simulink model "FMS"  (R2018b)
settings: configuration reference "fms_config" (kept outside this file)
values from neighbouring files (symbols this model uses):
  FMS_EXPORT = Simulink.Parameter(FMS_EXPORT_VALUE)    [fms_model_init.m]
  FMS_PARAM = Simulink.Parameter(FMS_PARAM_VALUE)    [fms_model_init.m]
undefined symbols (not defined in the file or in its folder): actuator_cmd, ax_cmd, ay_cmd, az_cmd, cmd_mask, ControlMode, ctrl_mode, DiscIntNeverNeededParam, ext_state, FMS_Cmd, FMS_CONST, home, mode, p_cmd, phi_cmd, PilotMode, psi_rate_cmd, q_cmd, r_cmd, reset, state, status, theta_cmd, throttle_cmd, timestamp, u_cmd, v_cmd, VehicleState, VehicleStatus, VTOLState, w_cmd, wp_consume, wp_current
libraries: simulink x141, FMT_Model_Lib x120, hdlsllib x13
(part 8 of 12)

== system FMS/FMS Commander/Commander/Arm/MC_Mode/SubMode/Takeoff/Climb Speed/TD/fhan  ==
  v1 : Inport
  v2 : Inport  Port=2
  Abs : Abs
  Add{,1..3,5..6} (6 alike) : Sum  OutDataTypeStr=Inherit: Same as first input
  Add4 : Sum  Inputs=-++
  Divide : Product  Inputs=*/
  Gain : Gain  Gain=8
  Gain1 : Gain  Gain=0.5  OutDataTypeStr=Inherit: Same as input
  Gain2 : Gain  Gain=0.5  OutDataTypeStr=Inherit: Same as input
  Gain3 : Gain  Gain=0.5  OutDataTypeStr=Inherit: Same as input
  Gain4 : Gain  Gain=-1  OutDataTypeStr=Inherit: Same as input
  Multiply{,1..3} (4 alike) : Product  OutDataTypeStr=Inherit: Same as first input
  Multiply4 : Product  OutDataTypeStr=single
  Multiply5 : Product  Inputs=3
  Multiply6 : Product  OutDataTypeStr=single
  Sign{,1..6} (7 alike) : Signum
  Sqrt : Sqrt  SaturateOnIntegerOverflow=on
  Square : Math  Operator=square  SaturateOnIntegerOverflow=on
  Subtract{,1..5} (6 alike) : Sum  Inputs=+-  OutDataTypeStr=Inherit: Same as first input
  Subtract6 : Sum  Inputs=-+  OutDataTypeStr=Inherit: Same as first input
  const : Constant  Value=r0  OutDataTypeStr=single
  const1 : Constant  Value=h0  OutDataTypeStr=single
  fhan : Outport
  wires:
  v1/1 -> Add/1
  Sign/1 -> Multiply3/1
  Gain2/1 -> Multiply4/2  "sy"
  v2/1 -> Multiply1/1
  Gain3/1 -> Multiply5/3  "sa"
  Subtract/1 -> Gain1/1
  Subtract6/1 -> fhan/1
  Sign2/1 -> Subtract2/2
  Sign4/1 -> Subtract4/2
  Abs/1 -> Gain/1
  Add4/1 -> Multiply4/1
  Sign5/1 -> Subtract5/2
  Sqrt/1 -> Subtract/1  "a1"
  Subtract3/1 -> Sign4/1
  Add1/1 -> Multiply2/1
  Subtract1/1 -> Sign2/1
  Divide/1 -> Subtract5/1
  Multiply3/1 -> Add2/1
  Gain/1 -> Add1/2
  const/1 -> Multiply6/2, Gain4/1, Multiply/1
  Add3/1 -> Sign1/1
  Subtract5/1 -> Multiply5/2
  Multiply4/1 -> Add5/2
  const1/1 -> Multiply1/2, Square/1
  Add5/1 -> Sign6/1, Sign5/1, Divide/1, Subtract3/1, Add6/1  "a"
  Multiply1/1 -> Add4/3, Add2/2, Add/2  "a0"
  Add/1 -> Subtract1/1, Add3/1, Add4/2, Sign/1, Abs/1  "y"
  Subtract2/1 -> Gain2/1
  Add2/1 -> Add4/1, Add5/1  "a2"
  Subtract4/1 -> Gain3/1
  Gain4/1 -> Multiply5/1
  Multiply5/1 -> Subtract6/2
  Sign6/1 -> Multiply6/1
  Sign3/1 -> Subtract4/1
  Add6/1 -> Sign3/1
  Multiply/1 -> Subtract/2, Divide/2, Subtract3/2, Add6/2, Subtract1/2, Add3/2, Add1/1, Multiply2/2  "d"
  Multiply6/1 -> Subtract6/1
  Gain1/1 -> Multiply3/2
  Square/1 -> Multiply/2
  Multiply2/1 -> Sqrt/1
  Sign1/1 -> Subtract2/1

== system FMS/FMS Commander/Commander/Arm/BackwardTrans_Mode/Position Command/Controller/Hold Control/Lateral_Acceleration/L1_Lateral_Acceleration/Included Angle ==
  vec1 : Inport
  vec2 : Inport  Port=2
  2D Cross Product : FMT_Model_Lib/Math/2D Cross Product
      settings: SourceProductName=FMT Toolbox
  Acos : Trigonometry  Operator=acos
  Constant4 : Constant  OutDataTypeStr=single
  Demux : Demux  Outputs=2
  Demux1 : Demux  Outputs=2
  Dot Product : DotProduct  InputSameDT=on  OutDataTypeStr=Inherit: Inherit via internal rule
  Multiply : Product
  Mux : Mux  Inputs=2
  Mux1 : Mux  Inputs=2
  Sign1 : Signum
  Switch2 : Switch  Criteria=u2 ~= 0
  Vector Normalize : FMT_Model_Lib/Math/Vector Normalize
      settings: SourceProductName=FMT Toolbox
  Vector Normalize1 : FMT_Model_Lib/Math/Vector Normalize
      settings: SourceProductName=FMT Toolbox
  angle_rad : Outport
  wires:
  Switch2/1 -> Multiply/2
  Acos/1 -> Multiply/1
  Mux/1 -> Vector Normalize1/1
  vec2/1 -> Demux/1
  Constant4/1 -> Switch2/3
  Demux/1 -> Mux/2
  vec1/1 -> Demux1/1
  Multiply/1 -> angle_rad/1
  2D Cross Product/1 -> Sign1/1
  Vector Normalize/1 -> 2D Cross Product/2, Dot Product/1
  Demux/2 -> Mux/1
  Vector Normalize1/1 -> 2D Cross Product/1, Dot Product/2
  Sign1/1 -> Switch2/2, Switch2/1
  Demux1/2 -> Mux1/1
  Mux1/1 -> Vector Normalize/1
  Demux1/1 -> Mux1/2
  Dot Product/1 -> Acos/1

== system FMS/FMS Commander/Commander/Arm/BackwardTrans_Mode/Position Command/Controller/Hold Control/Velocity_Controller/Error/Bus_Select ==
  INS_Out : Inport
  Bus Selector1 : BusSelector  OutputSignals=vn,ve
  Bus Selector2 : BusSelector  OutputSignals=psi
  Constant : Constant  Value=0  OutDataTypeStr=single
  Multiply : Product  Multiplication=Matrix(*)
  Mux2 : Mux  Inputs=3
  Psi To DCM : FMT_Model_Lib/Transformation/Psi To DCM
      settings: SourceProductName=FMT Toolbox
  Selector : Selector  InputPortWidth=3  IndexOptions=Index vector (dialog)  Indices=2  OutputSizes=1
  v_est_C_mPs : Outport
  wires:
  Psi To DCM/1 -> Multiply/1
  Bus Selector2/1 -> Psi To DCM/1  "<psi>"
  Constant/1 -> Mux2/3  "<velD>"
  Mux2/1 -> Multiply/2
  Bus Selector1/2 -> Mux2/2  "<ve>"
  Bus Selector1/1 -> Mux2/1  "<vn>"
  INS_Out/1 -> Bus Selector2/1, Bus Selector1/1
  Multiply/1 -> Selector/1
  Selector/1 -> v_est_C_mPs/1

== system FMS/FMS Commander/Commander/Arm/BackwardTrans_Mode/Position Command/Controller/Hold Control/Velocity_Controller/PID_Controller/D_Control ==
  err : Inport
  reset : Inport  Port=2
  DT Filter : FMT_Model_Lib/Filter/DT Filter  fc=10
      settings: SourceProductName=FMT Toolbox
  Multiply : Product  OutDataTypeStr=Inherit: Same as first input
  Saturation : Saturate  UpperLimit=max_d  LowerLimit=min_d
  kd : Constant  Value=kd  OutDataTypeStr=single
  d_out : Outport
  wires:
  err/1 -> DT Filter/1
  kd/1 -> Multiply/1
  Multiply/1 -> Saturation/1
  Saturation/1 -> d_out/1
  reset/1 -> DT Filter/2
  DT Filter/1 -> Multiply/2

== system FMS/FMS Commander/Commander/Arm/BackwardTrans_Mode/Position Command/Controller/Hold Control/Velocity_Controller/PID_Controller/I_Control ==
  err : Inport
  reset : Inport  Port=2
  Constant : Constant  Value=0  OutDataTypeStr=single
  Discrete-Time Integrator : DiscreteIntegrator  ExternalReset=level  InitialConditionSource=external  SampleTime=-1  LimitOutput=on  UpperSaturationLimit=max_i  LowerSaturationLimit=min_i  ICPrevOutput=DiscIntNeverNeededParam  ICPrevScaledInput=DiscIntNeverNeededParam
  Multiply : Product  OutDataTypeStr=Inherit: Same as first input
  ki : Constant  Value=ki  OutDataTypeStr=single
  i_out : Outport
  wires:
  err/1 -> Multiply/2
  Multiply/1 -> Discrete-Time Integrator/1
  reset/1 -> Discrete-Time Integrator/2
  Constant/1 -> Discrete-Time Integrator/3
  Discrete-Time Integrator/1 -> i_out/1
  ki/1 -> Multiply/1

== system FMS/FMS Commander/Commander/Arm/BackwardTrans_Mode/Position Command/Controller/Hold Control/Velocity_Controller/PID_Controller/P_Control ==
  err : Inport
  Multiply : Product  OutDataTypeStr=Inherit: Same as first input
  kp : Constant  Value=kp  OutDataTypeStr=single
  p_out : Outport
  wires:
  err/1 -> Multiply/2
  kp/1 -> Multiply/1
  Multiply/1 -> p_out/1

== system FMS/FMS Commander/Commander/Arm/FW_Mode/Assist/Altitude/Altitude Command/Controller/Hold Control/Bus_Selection ==
  FMS_In : Inport
  Bus Selector2 : BusSelector  OutputSignals=INS_Out.h_R
  Gain : Gain  Gain=-1
  z_R_m : Outport
  wires:
  Gain/1 -> z_R_m/1
  Bus Selector2/1 -> Gain/1  "<h_R>"
  FMS_In/1 -> Bus Selector2/1

== system FMS/FMS Commander/Commander/Arm/FW_Mode/Assist/Altitude/Altitude Command/Controller/Move Control/DeadZone ==
  u : Inport
  Dead Zone : DeadZone  LowerValue=-th  UpperValue=th  SaturateOnIntegerOverflow=on
  Gain : Gain  Gain=1/(1-th)
  y : Outport
  wires:
  Gain/1 -> y/1
  Dead Zone/1 -> Gain/1
  u/1 -> Dead Zone/1

== system FMS/FMS Commander/Commander/Arm/FW_Mode/Assist/Altitude/Altitude Command/Controller/Move Control/TD1 ==
  v : Inport
  Integrator : DiscreteIntegrator  SampleTime=-1  ICPrevOutput=DiscIntNeverNeededParam  ICPrevScaledInput=DiscIntNeverNeededParam
  Integrator1 : DiscreteIntegrator  SampleTime=-1  ICPrevOutput=DiscIntNeverNeededParam  ICPrevScaledInput=DiscIntNeverNeededParam
  Subtract : Sum  Inputs=+-
  "fhan " : Subsystem  mask{r0=8*9.806, h0=0.05}
      mask DialogControl ParameterGroupVar Prompt: fhan(v1,v2,r0,h0)
  v1 : Outport
  wires:
  Integrator1/1 -> v1/1, Subtract/1
  v/1 -> Subtract/2
  Integrator/1 -> "fhan "/2(v2), Integrator1/1  "v2"
  Subtract/1 -> "fhan "/1(v1)
  "fhan "/1(fhan) -> Integrator/1

== system FMS/FMS Commander/Commander/Arm/FW_Mode/Assist/Altitude/Altitude Command/Controller/TD/fhan  ==
  v1 : Inport
  v2 : Inport  Port=2
  Abs : Abs
  Add{,1..3,5..6} (6 alike) : Sum  OutDataTypeStr=Inherit: Same as first input
  Add4 : Sum  Inputs=-++
  Divide : Product  Inputs=*/
  Gain : Gain  Gain=8
  Gain1 : Gain  Gain=0.5  OutDataTypeStr=Inherit: Same as input
  Gain2 : Gain  Gain=0.5  OutDataTypeStr=Inherit: Same as input
  Gain3 : Gain  Gain=0.5  OutDataTypeStr=Inherit: Same as input
  Gain4 : Gain  Gain=-1  OutDataTypeStr=Inherit: Same as input
  Multiply{,1..3} (4 alike) : Product  OutDataTypeStr=Inherit: Same as first input
  Multiply4 : Product  OutDataTypeStr=single
  Multiply5 : Product  Inputs=3
  Multiply6 : Product  OutDataTypeStr=single
  Sign{,1..6} (7 alike) : Signum
  Sqrt : Sqrt  SaturateOnIntegerOverflow=on
  Square : Math  Operator=square  SaturateOnIntegerOverflow=on
  Subtract{,1..5} (6 alike) : Sum  Inputs=+-  OutDataTypeStr=Inherit: Same as first input
  Subtract6 : Sum  Inputs=-+  OutDataTypeStr=Inherit: Same as first input
  const : Constant  Value=r0  OutDataTypeStr=single
  const1 : Constant  Value=h0  OutDataTypeStr=single
  fhan : Outport
  wires:
  Sign1/1 -> Subtract2/1
  Multiply2/1 -> Sqrt/1
  Square/1 -> Multiply/2
  Gain1/1 -> Multiply3/2
  Multiply6/1 -> Subtract6/1
  Multiply/1 -> Multiply2/2, Add1/1, Add3/2, Subtract1/2, Add6/2, Subtract3/2, Divide/2, Subtract/2  "d"
  Add6/1 -> Sign3/1
  Sign3/1 -> Subtract4/1
  Sign6/1 -> Multiply6/1
  Multiply5/1 -> Subtract6/2
  Gain4/1 -> Multiply5/1
  Subtract4/1 -> Gain3/1
  Add2/1 -> Add5/1, Add4/1  "a2"
  Subtract2/1 -> Gain2/1
  Add/1 -> Abs/1, Sign/1, Add4/2, Add3/1, Subtract1/1  "y"
  Multiply1/1 -> Add/2, Add2/2, Add4/3  "a0"
  Add5/1 -> Add6/1, Subtract3/1, Divide/1, Sign5/1, Sign6/1  "a"
  const1/1 -> Square/1, Multiply1/2
  Multiply4/1 -> Add5/2
  Subtract5/1 -> Multiply5/2
  Add3/1 -> Sign1/1
  const/1 -> Multiply/1, Gain4/1, Multiply6/2
  Gain/1 -> Add1/2
  Multiply3/1 -> Add2/1
  Divide/1 -> Subtract5/1
  Subtract1/1 -> Sign2/1
  Add1/1 -> Multiply2/1
  Subtract3/1 -> Sign4/1
  Sqrt/1 -> Subtract/1  "a1"
  Sign5/1 -> Subtract5/2
  Add4/1 -> Multiply4/1
  Abs/1 -> Gain/1
  Sign4/1 -> Subtract4/2
  Sign2/1 -> Subtract2/2
  Subtract6/1 -> fhan/1
  Subtract/1 -> Gain1/1
  Gain3/1 -> Multiply5/3  "sa"
  v2/1 -> Multiply1/1
  Gain2/1 -> Multiply4/2  "sy"
  Sign/1 -> Multiply3/1
  v1/1 -> Add/1

== system FMS/FMS Commander/Commander/Arm/FW_Mode/Assist/Position/Altitude Command/Controller/Hold Control/Bus_Selection ==
  FMS_In : Inport
  Bus Selector2 : BusSelector  OutputSignals=INS_Out.h_R
  Gain : Gain  Gain=-1
  z_R_m : Outport
  wires:
  Gain/1 -> z_R_m/1
  Bus Selector2/1 -> Gain/1  "<h_R>"
  FMS_In/1 -> Bus Selector2/1

== system FMS/FMS Commander/Commander/Arm/FW_Mode/Assist/Position/Altitude Command/Controller/Move Control/DeadZone ==
  u : Inport
  Dead Zone : DeadZone  LowerValue=-th  UpperValue=th  SaturateOnIntegerOverflow=on
  Gain : Gain  Gain=1/(1-th)
  y : Outport
  wires:
  Gain/1 -> y/1
  Dead Zone/1 -> Gain/1
  u/1 -> Dead Zone/1

== system FMS/FMS Commander/Commander/Arm/FW_Mode/Assist/Position/Altitude Command/Controller/Move Control/TD1 ==
  v : Inport
  Integrator : DiscreteIntegrator  SampleTime=-1  ICPrevOutput=DiscIntNeverNeededParam  ICPrevScaledInput=DiscIntNeverNeededParam
  Integrator1 : DiscreteIntegrator  SampleTime=-1  ICPrevOutput=DiscIntNeverNeededParam  ICPrevScaledInput=DiscIntNeverNeededParam
  Subtract : Sum  Inputs=+-
  "fhan " : Subsystem  mask{r0=8*9.806, h0=0.05}
      mask DialogControl ParameterGroupVar Prompt: fhan(v1,v2,r0,h0)
  v1 : Outport
  wires:
  Integrator1/1 -> v1/1, Subtract/1
  v/1 -> Subtract/2
  Integrator/1 -> "fhan "/2(v2), Integrator1/1  "v2"
  Subtract/1 -> "fhan "/1(v1)
  "fhan "/1(fhan) -> Integrator/1

== system FMS/FMS Commander/Commander/Arm/FW_Mode/Assist/Position/Altitude Command/Controller/TD/fhan  ==
  v1 : Inport
  v2 : Inport  Port=2
  Abs : Abs
  Add{,1..3,5..6} (6 alike) : Sum  OutDataTypeStr=Inherit: Same as first input
  Add4 : Sum  Inputs=-++
  Divide : Product  Inputs=*/
  Gain : Gain  Gain=8
  Gain1 : Gain  Gain=0.5  OutDataTypeStr=Inherit: Same as input
  Gain2 : Gain  Gain=0.5  OutDataTypeStr=Inherit: Same as input
  Gain3 : Gain  Gain=0.5  OutDataTypeStr=Inherit: Same as input
  Gain4 : Gain  Gain=-1  OutDataTypeStr=Inherit: Same as input
  Multiply{,1..3} (4 alike) : Product  OutDataTypeStr=Inherit: Same as first input
  Multiply4 : Product  OutDataTypeStr=single
  Multiply5 : Product  Inputs=3
  Multiply6 : Product  OutDataTypeStr=single
  Sign{,1..6} (7 alike) : Signum
  Sqrt : Sqrt  SaturateOnIntegerOverflow=on
  Square : Math  Operator=square  SaturateOnIntegerOverflow=on
  Subtract{,1..5} (6 alike) : Sum  Inputs=+-  OutDataTypeStr=Inherit: Same as first input
  Subtract6 : Sum  Inputs=-+  OutDataTypeStr=Inherit: Same as first input
  const : Constant  Value=r0  OutDataTypeStr=single
  const1 : Constant  Value=h0  OutDataTypeStr=single
  fhan : Outport
  wires:
  Sign1/1 -> Subtract2/1
  Multiply2/1 -> Sqrt/1
  Square/1 -> Multiply/2
  Gain1/1 -> Multiply3/2
  Multiply6/1 -> Subtract6/1
  Multiply/1 -> Multiply2/2, Add1/1, Add3/2, Subtract1/2, Add6/2, Subtract3/2, Divide/2, Subtract/2  "d"
  Add6/1 -> Sign3/1
  Sign3/1 -> Subtract4/1
  Sign6/1 -> Multiply6/1
  Multiply5/1 -> Subtract6/2
  Gain4/1 -> Multiply5/1
  Subtract4/1 -> Gain3/1
  Add2/1 -> Add5/1, Add4/1  "a2"
  Subtract2/1 -> Gain2/1
  Add/1 -> Abs/1, Sign/1, Add4/2, Add3/1, Subtract1/1  "y"
  Multiply1/1 -> Add/2, Add2/2, Add4/3  "a0"
  Add5/1 -> Add6/1, Subtract3/1, Divide/1, Sign5/1, Sign6/1  "a"
  const1/1 -> Square/1, Multiply1/2
  Multiply4/1 -> Add5/2
  Subtract5/1 -> Multiply5/2
  Add3/1 -> Sign1/1
  const/1 -> Multiply/1, Gain4/1, Multiply6/2
  Gain/1 -> Add1/2
  Multiply3/1 -> Add2/1
  Divide/1 -> Subtract5/1
  Subtract1/1 -> Sign2/1
  Add1/1 -> Multiply2/1
  Subtract3/1 -> Sign4/1
  Sqrt/1 -> Subtract/1  "a1"
  Sign5/1 -> Subtract5/2
  Add4/1 -> Multiply4/1
  Abs/1 -> Gain/1
  Sign4/1 -> Subtract4/2
  Sign2/1 -> Subtract2/2
  Subtract6/1 -> fhan/1
  Subtract/1 -> Gain1/1
  Gain3/1 -> Multiply5/3  "sa"
  v2/1 -> Multiply1/1
  Gain2/1 -> Multiply4/2  "sy"
  Sign/1 -> Multiply3/1
  v1/1 -> Add/1

== system FMS/FMS Commander/Commander/Arm/FW_Mode/Assist/Position/Position Command/Controller/Hold Control/Fly_Direction ==
  FMS_In : Inport
  Bus Selector2 : BusSelector  OutputSignals=INS_Out.vn,INS_Out.ve,INS_Out.vd
  Bus Selector3 : BusSelector  OutputSignals=INS_Out.quat
  Multiply : Product  Multiplication=Matrix(*)
  Mux : Mux  Inputs=3
  Quaternion To DCM : FMT_Model_Lib/Quaternion/Quaternion To DCM
      settings: SourceProductName=FMT Toolbox
  Selector : Selector  InputPortWidth=3  IndexOptions=Index vector (dialog)  Indices=1  OutputSizes=1
  Sign : Signum
  sign : Outport
  wires:
  Bus Selector3/1 -> Quaternion To DCM/1  "<quat>"
  Multiply/1 -> Selector/1
  Bus Selector2/3 -> Mux/3  "<vd>"
  FMS_In/1 -> Bus Selector3/1, Bus Selector2/1
  Sign/1 -> sign/1
  Mux/1 -> Multiply/2
  Quaternion To DCM/1 -> Multiply/1
  Bus Selector2/2 -> Mux/2  "<ve>"
  Bus Selector2/1 -> Mux/1  "<vn>"
  Selector/1 -> Sign/1  "Vu"

== system FMS/FMS Commander/Commander/Arm/FW_Mode/Assist/Position/Position Command/Controller/Hold Control/L1_Reference_WP ==
  c : Inport
  p_0 : Inport  Port=2
  n : Inport  Port=3
  L1 : Inport  Port=4
  Compare To Zero : simulink/Logic and Bit Operations/Compare To Zero  relop=>  OutDataTypeStr=boolean
  OutRegionRefWP : MATLAB Function  TreatAsAtomicUnit=on
  SearchL1RefWP : MATLAB Function  TreatAsAtomicUnit=on
  Switch : Switch  Criteria=u2 > Threshold
  L1_WP : Outport
  wires:
  c/1 -> OutRegionRefWP/1(c), SearchL1RefWP/1(c)
  p_0/1 -> OutRegionRefWP/2(p0), SearchL1RefWP/2(p0)
  n/1 -> OutRegionRefWP/3(n), SearchL1RefWP/3(n)
  L1/1 -> SearchL1RefWP/4(L1)
  SearchL1RefWP/1(P) -> Switch/1
  SearchL1RefWP/2(t) -> Compare To Zero/1
  Compare To Zero/1 -> Switch/2
  OutRegionRefWP/1(P) -> Switch/3
  Switch/1 -> L1_WP/1

== system FMS/FMS Commander/Commander/Arm/FW_Mode/Assist/Position/Position Command/Controller/Hold Control/Lateral_Acceleration ==
  p_vehicle : Inport
  L1_WP : Inport  Port=2
  L1 : Inport  Port=3
  Vg : Inport  Port=4
  L1_Lateral_Acceleration : Subsystem
  Subtract : Sum  Inputs=+-
  ay_cmd_mPs2 : Outport
  wires:
  L1_WP/1 -> Subtract/1
  p_vehicle/1 -> Subtract/2
  L1/1 -> L1_Lateral_Acceleration/1(L1)
  Vg/1 -> L1_Lateral_Acceleration/2(Vg)
  Subtract/1 -> L1_Lateral_Acceleration/3(l1_path)
  L1_Lateral_Acceleration/1(l1_a_cmd) -> ay_cmd_mPs2/1

== system FMS/FMS Commander/Commander/Arm/FW_Mode/Assist/Position/Position Command/Controller/Hold Control/Path_Ray ==
  note: p(t) = p0 + t*n
  FMS_In : Inport
  Bus Selector1 : BusSelector  OutputSignals=INS_Out.x_R,INS_Out.y_R
  Bus Selector2 : BusSelector  OutputSignals=INS_Out.vn,INS_Out.ve
  Bus Selector3 : BusSelector  Commented=on  OutputSignals=INS_Out.psi
  Constant : Constant  Commented=on  Value=[1;0;0]  VectorParams1D=off  OutDataTypeStr=single
  Multiply : Product  Commented=on  Multiplication=Matrix(*)
  Mux : Mux  Inputs=2
  Mux1 : Mux  Inputs=2
  Psi To DCM : FMT_Model_Lib/Transformation/Psi To DCM  Commented=on
      settings: SourceProductName=FMT Toolbox
  Selector : Selector  Commented=on  InputPortWidth=3  IndexOptions=Index vector (dialog)  Indices=[1 2]  OutputSizes=1
  Terminator : Terminator  Commented=on
  Transpose : Math  Commented=on  Operator=transpose  SaturateOnIntegerOverflow=on
  Vector Normalize : FMT_Model_Lib/Math/Vector Normalize
      settings: SourceProductName=FMT Toolbox
  start_vel : Delay  DelayLength=1  InitialConditionSource=Input port
      settings: InputPortMap=u0,p4
  start_wp : Delay  DelayLength=1  InitialConditionSource=Input port
      settings: InputPortMap=u0,p4
  p_vehicle : Outport
  p_0 : Outport  Port=2
  n : Outport  Port=3
  wires:
  Bus Selector2/2 -> Mux1/2  "<ve>"
  Bus Selector1/2 -> Mux/2  "<y_R>"
  Mux/1 -> p_vehicle/1, start_wp/2
  start_wp/1 -> p_0/1, start_wp/1
  Bus Selector1/1 -> Mux/1  "<x_R>"
  start_vel/1 -> Vector Normalize/1, start_vel/1
  Bus Selector2/1 -> Mux1/1  "<vn>"
  Vector Normalize/1 -> n/1
  FMS_In/1 -> Bus Selector3/1, Bus Selector2/1, Bus Selector1/1
  Mux1/1 -> start_vel/2
  Bus Selector3/1 -> Psi To DCM/1  "<psi>"
  Psi To DCM/1 -> Transpose/1
  Transpose/1 -> Multiply/1
  Constant/1 -> Multiply/2
  Multiply/1 -> Selector/1
  Selector/1 -> Terminator/1

== system FMS/FMS Commander/Commander/Arm/FW_Mode/Assist/Position/Position Command/Controller/Hold Control/Velocity_Controller ==
  FMS_In : Inport
  Bus Selector : BusSelector  OutputSignals=INS_Out
  Constant : Constant  Value=0  OutDataTypeStr=Inherit: Inherit via back propagation
  Error : Subsystem
  PID_Controller : Subsystem
  ay_cmd_B_rad : Outport
  wires:
  FMS_In/1 -> Bus Selector/1
  Error/1(v_err_C_mPs) -> PID_Controller/1(uv_err_C_mPs)
  PID_Controller/1(accel_cmd_C) -> ay_cmd_B_rad/1
  Bus Selector/1 -> Error/1(INS_Out)  "<INS_Out>"
  Constant/1 -> PID_Controller/2(reset)

== system FMS/FMS Commander/Commander/Arm/FW_Mode/Assist/Position/Position Command/Controller/Move Control/DeadZone1 ==
  u : Inport
  Dead Zone : DeadZone  LowerValue=-th  UpperValue=th  SaturateOnIntegerOverflow=on
  Gain : Gain  Gain=1/(1-th)
  y : Outport
  wires:
  u/1 -> Dead Zone/1
  Dead Zone/1 -> Gain/1
  Gain/1 -> y/1

== system FMS/FMS Commander/Commander/Arm/FW_Mode/Assist/Position/Position Command/Controller/Move Control/TD ==
  v : Inport
  Integrator : DiscreteIntegrator  SampleTime=-1  ICPrevOutput=DiscIntNeverNeededParam  ICPrevScaledInput=DiscIntNeverNeededParam
  Integrator1 : DiscreteIntegrator  SampleTime=-1  ICPrevOutput=DiscIntNeverNeededParam  ICPrevScaledInput=DiscIntNeverNeededParam
  Subtract : Sum  Inputs=+-
  "fhan " : Subsystem  mask{r0=6*9.806, h0=0.05}
      mask DialogControl ParameterGroupVar Prompt: fhan(v1,v2,r0,h0)
  v1 : Outport
  wires:
  "fhan "/1(fhan) -> Integrator/1
  Subtract/1 -> "fhan "/1(v1)
  Integrator/1 -> Integrator1/1, "fhan "/2(v2)  "v2"
  v/1 -> Subtract/2
  Integrator1/1 -> Subtract/1, v1/1

== system FMS/FMS Commander/Commander/Arm/FW_Mode/Auto/Mission/Mission_SubSystem/Cruise_Speed/TD/fhan  ==
  v1 : Inport
  v2 : Inport  Port=2
  Abs : Abs
  Add{,1..3,5..6} (6 alike) : Sum  OutDataTypeStr=Inherit: Same as first input
  Add4 : Sum  Inputs=-++
  Divide : Product  Inputs=*/
  Gain : Gain  Gain=8
  Gain1 : Gain  Gain=0.5  OutDataTypeStr=Inherit: Same as input
  Gain2 : Gain  Gain=0.5  OutDataTypeStr=Inherit: Same as input
  Gain3 : Gain  Gain=0.5  OutDataTypeStr=Inherit: Same as input
  Gain4 : Gain  Gain=-1  OutDataTypeStr=Inherit: Same as input
  Multiply{,1..3} (4 alike) : Product  OutDataTypeStr=Inherit: Same as first input
  Multiply4 : Product  OutDataTypeStr=single
  Multiply5 : Product  Inputs=3
  Multiply6 : Product  OutDataTypeStr=single
  Sign{,1..6} (7 alike) : Signum
  Sqrt : Sqrt  SaturateOnIntegerOverflow=on
  Square : Math  Operator=square  SaturateOnIntegerOverflow=on
  Subtract{,1..5} (6 alike) : Sum  Inputs=+-  OutDataTypeStr=Inherit: Same as first input
  Subtract6 : Sum  Inputs=-+  OutDataTypeStr=Inherit: Same as first input
  const : Constant  Value=r0  OutDataTypeStr=single
  const1 : Constant  Value=h0  OutDataTypeStr=single
  fhan : Outport
  wires:
  Sign1/1 -> Subtract2/1
  Multiply2/1 -> Sqrt/1
  Square/1 -> Multiply/2
  Gain1/1 -> Multiply3/2
  Multiply6/1 -> Subtract6/1
  Multiply/1 -> Multiply2/2, Add1/1, Add3/2, Subtract1/2, Add6/2, Subtract3/2, Divide/2, Subtract/2  "d"
  Add6/1 -> Sign3/1
  Sign3/1 -> Subtract4/1
  Sign6/1 -> Multiply6/1
  Multiply5/1 -> Subtract6/2
  Gain4/1 -> Multiply5/1
  Subtract4/1 -> Gain3/1
  Add2/1 -> Add5/1, Add4/1  "a2"
  Subtract2/1 -> Gain2/1
  Add/1 -> Abs/1, Sign/1, Add4/2, Add3/1, Subtract1/1  "y"
  Multiply1/1 -> Add/2, Add2/2, Add4/3  "a0"
  Add5/1 -> Add6/1, Subtract3/1, Divide/1, Sign5/1, Sign6/1  "a"
  const1/1 -> Square/1, Multiply1/2
  Multiply4/1 -> Add5/2
  Subtract5/1 -> Multiply5/2
  Add3/1 -> Sign1/1
  const/1 -> Multiply/1, Gain4/1, Multiply6/2
  Gain/1 -> Add1/2
  Multiply3/1 -> Add2/1
  Divide/1 -> Subtract5/1
  Subtract1/1 -> Sign2/1
  Add1/1 -> Multiply2/1
  Subtract3/1 -> Sign4/1
  Sqrt/1 -> Subtract/1  "a1"
  Sign5/1 -> Subtract5/2
  Add4/1 -> Multiply4/1
  Abs/1 -> Gain/1
  Sign4/1 -> Subtract4/2
  Sign2/1 -> Subtract2/2
  Subtract6/1 -> fhan/1
  Subtract/1 -> Gain1/1
  Gain3/1 -> Multiply5/3  "sa"
  v2/1 -> Multiply1/1
  Gain2/1 -> Multiply4/2  "sy"
  Sign/1 -> Multiply3/1
  v1/1 -> Add/1

== system FMS/FMS Commander/Commander/Arm/FW_Mode/Auto/Mission/Mission_SubSystem/Position Command/L1 Control/L1 Reference WP ==
  P1 : Inport
  P2 : Inport  Port=2
  P3 : Inport  Port=3
  L1 : Inport  Port=4
  Compare To Constant : simulink/Logic and Bit Operations/Compare To Constant  relop=>=  const=0  OutDataTypeStr=boolean
  Compare To Constant1 : simulink/Logic and Bit Operations/Compare To Constant  relop=>  const=0  OutDataTypeStr=boolean
  NearbyRefWP : MATLAB Function  TreatAsAtomicUnit=on
  OutRegionRegWP : MATLAB Function  TreatAsAtomicUnit=on
  Reshape : Reshape  OutputDimensionality=Customize  OutputDimensions=[2,1]
  SearchL1RefWP : MATLAB Function  TreatAsAtomicUnit=on
  Switch : Switch  Criteria=u2 > Threshold
  Switch1 : Switch  Criteria=u2 > Threshold
  L1_WP : Outport
  wires:
  Reshape/1 -> L1_WP/1
  Compare To Constant/1 -> Switch/2
  NearbyRefWP/2(d) -> Compare To Constant1/1  "distance"
  SearchL1RefWP/2(u) -> Compare To Constant/1  "l1_u"
  Compare To Constant1/1 -> Switch1/2
  P1/1 -> SearchL1RefWP/1(P1), OutRegionRegWP/1(P1)
  P2/1 -> SearchL1RefWP/2(P2), NearbyRefWP/1(P2), OutRegionRegWP/2(P2)
  P3/1 -> NearbyRefWP/2(P3), SearchL1RefWP/3(P3), OutRegionRegWP/3(P3)
  Switch/1 -> Switch1/3
  L1/1 -> OutRegionRegWP/4(L1), SearchL1RefWP/4(L1), NearbyRefWP/3(L1)
  OutRegionRegWP/1(P) -> Switch/3  "out_WP"
  Switch1/1 -> Reshape/1
  SearchL1RefWP/1(P) -> Switch/1  "L1_Ref_P"
  NearbyRefWP/1(P) -> Switch1/1  "NearbyWP"

== system FMS/FMS Commander/Commander/Arm/FW_Mode/Auto/Mission/Mission_SubSystem/Position Command/L1 Control/L1_Core ==
  p_vehicle : Inport
  L1_WP : Inport  Port=2
  L1 : Inport  Port=3
  Vg : Inport  Port=4
  L1_Lateral_Acceleration : Subsystem
  Subtract : Sum  Inputs=+-
  ay_cmd_mPs2 : Outport
  wires:
  L1_WP/1 -> Subtract/1
  p_vehicle/1 -> Subtract/2
  L1/1 -> L1_Lateral_Acceleration/1(L1)
  Vg/1 -> L1_Lateral_Acceleration/2(Vg)
  Subtract/1 -> L1_Lateral_Acceleration/3(l1_path)
  L1_Lateral_Acceleration/1(l1_a_cmd) -> ay_cmd_mPs2/1

== system FMS/FMS Commander/Commander/Arm/FW_Mode/SubMode/Hold/Loiter_Control/L1_Core/L1_Lateral_Acceleration/Included Angle ==
  vec1 : Inport
  vec2 : Inport  Port=2
  2D Cross Product : FMT_Model_Lib/Math/2D Cross Product
      settings: SourceProductName=FMT Toolbox
  Acos : Trigonometry  Operator=acos
  Constant4 : Constant  OutDataTypeStr=single
  Demux : Demux  Outputs=2
  Demux1 : Demux  Outputs=2
  Dot Product : DotProduct  InputSameDT=on  OutDataTypeStr=Inherit: Inherit via internal rule
  Multiply : Product
  Mux : Mux  Inputs=2
  Mux1 : Mux  Inputs=2
  Sign1 : Signum
  Switch2 : Switch  Criteria=u2 ~= 0
  Vector Normalize : FMT_Model_Lib/Math/Vector Normalize
      settings: SourceProductName=FMT Toolbox
  Vector Normalize1 : FMT_Model_Lib/Math/Vector Normalize
      settings: SourceProductName=FMT Toolbox
  angle_rad : Outport
  wires:
  Switch2/1 -> Multiply/2
  Acos/1 -> Multiply/1
  Mux/1 -> Vector Normalize1/1
  vec2/1 -> Demux/1
  Constant4/1 -> Switch2/3
  Demux/1 -> Mux/2
  vec1/1 -> Demux1/1
  Multiply/1 -> angle_rad/1
  2D Cross Product/1 -> Sign1/1
  Vector Normalize/1 -> 2D Cross Product/2, Dot Product/1
  Demux/2 -> Mux/1
  Vector Normalize1/1 -> 2D Cross Product/1, Dot Product/2
  Sign1/1 -> Switch2/2, Switch2/1
  Demux1/2 -> Mux1/1
  Mux1/1 -> Vector Normalize/1
  Demux1/1 -> Mux1/2
  Dot Product/1 -> Acos/1

== system FMS/FMS Commander/Commander/Arm/FW_Mode/SubMode/Return/Position Command/L1 Control/L1_Core/L1_Lateral_Acceleration ==
  L1 : Inport
  Vg : Inport  Port=2
  l1_path : Inport  Port=3
  Divide : Product  Inputs=*/
  Gain : Gain  Gain=2
  Included Angle : Subsystem
  Multiply1 : Product
  Saturation : Saturate  UpperLimit=pi/2  LowerLimit=-pi/2
  Sin : Trigonometry
  Square : Math  Operator=square  SaturateOnIntegerOverflow=on
  Vector Modulus : FMT_Model_Lib/Math/Vector Modulus
      settings: SourceProductName=FMT Toolbox
  Vector Normalize : FMT_Model_Lib/Math/Vector Normalize
      settings: SourceProductName=FMT Toolbox
  Vector Normalize1 : FMT_Model_Lib/Math/Vector Normalize
      settings: SourceProductName=FMT Toolbox
  l1_a_cmd : Outport
  wires:
  Vector Normalize/1 -> Included Angle/1(vec1)
  Included Angle/1(angle_rad) -> Saturation/1  "L1_alpha"
  Multiply1/1 -> Divide/1
  Divide/1 -> l1_a_cmd/1  "l1_a_cmd"
  Vector Normalize1/1 -> Included Angle/2(vec2)
  Sin/1 -> Multiply1/1  "sin_alpha"
  l1_path/1 -> Vector Normalize1/1
  Saturation/1 -> Sin/1
  Vg/1 -> Vector Normalize/1, Vector Modulus/1
  Square/1 -> Gain/1
  Gain/1 -> Multiply1/2
  L1/1 -> Divide/2
  Vector Modulus/1 -> Square/1

== system FMS/FMS Commander/Commander/Arm/FW_Mode/SubMode/Takeoff/Position Command/L1 Control/L1_Core/L1_Lateral_Acceleration ==
  L1 : Inport
  Vg : Inport  Port=2
  l1_path : Inport  Port=3
  Divide : Product  Inputs=*/
  Gain : Gain  Gain=2
  Included Angle : Subsystem
  Multiply1 : Product
  Saturation : Saturate  UpperLimit=pi/2  LowerLimit=-pi/2
  Sin : Trigonometry
  Square : Math  Operator=square  SaturateOnIntegerOverflow=on
  Vector Modulus : FMT_Model_Lib/Math/Vector Modulus
      settings: SourceProductName=FMT Toolbox
  Vector Normalize : FMT_Model_Lib/Math/Vector Normalize
      settings: SourceProductName=FMT Toolbox
  Vector Normalize1 : FMT_Model_Lib/Math/Vector Normalize
      settings: SourceProductName=FMT Toolbox
  l1_a_cmd : Outport
  wires:
  Vector Normalize/1 -> Included Angle/1(vec1)
  Included Angle/1(angle_rad) -> Saturation/1  "L1_alpha"
  Multiply1/1 -> Divide/1
  Divide/1 -> l1_a_cmd/1  "l1_a_cmd"
  Vector Normalize1/1 -> Included Angle/2(vec2)
  Sin/1 -> Multiply1/1  "sin_alpha"
  l1_path/1 -> Vector Normalize1/1
  Saturation/1 -> Sin/1
  Vg/1 -> Vector Normalize/1, Vector Modulus/1
  Square/1 -> Gain/1
  Gain/1 -> Multiply1/2
  L1/1 -> Divide/2
  Vector Modulus/1 -> Square/1

== system FMS/FMS Commander/Commander/Arm/MC_Mode/Assist/Altitude/Altitude Command/Controller/Hold Control/Bus_Selection ==
  FMS_In : Inport
  Bus Selector2 : BusSelector  OutputSignals=INS_Out.h_R
  Gain : Gain  Gain=-1
  z_R_m : Outport
  wires:
  Gain/1 -> z_R_m/1
  Bus Selector2/1 -> Gain/1  "<h_R>"
  FMS_In/1 -> Bus Selector2/1

== system FMS/FMS Commander/Commander/Arm/MC_Mode/Assist/Altitude/Altitude Command/Controller/Move Control/Assist Land Speed ==
  u : Inport
  Gain : Gain  Gain=0.5
  Land_Speed : Constant  Value=FMS_PARAM.LAND_SPEED  OutDataTypeStr=single
  Min : MinMax  Inputs=2
  y : Outport
  wires:
  u/1 -> Min/2
  Land_Speed/1 -> Min/1
  Min/1 -> Gain/1
  Gain/1 -> y/1

== system FMS/FMS Commander/Commander/Arm/MC_Mode/Assist/Altitude/Altitude Command/Controller/Move Control/DeadZone ==
  u : Inport
  Dead Zone : DeadZone  LowerValue=-th  UpperValue=th  SaturateOnIntegerOverflow=on
  Gain : Gain  Gain=1/(1-th)
  y : Outport
  wires:
  Gain/1 -> y/1
  Dead Zone/1 -> Gain/1
  u/1 -> Dead Zone/1

== system FMS/FMS Commander/Commander/Arm/MC_Mode/Assist/Altitude/Heading Command/Controller/Hold Control/Bus_Selection ==
  FMS_In : Inport
  Bus Selector2 : BusSelector  OutputSignals=INS_Out.psi
  psi_rad : Outport
  wires:
  Bus Selector2/1 -> psi_rad/1  "<psi>"
  FMS_In/1 -> Bus Selector2/1

== system FMS/FMS Commander/Commander/Arm/MC_Mode/Assist/Altitude/Heading Command/Controller/Hold Control/psi_err_saturation ==
  psi_err_in : Inport
  Abs : Abs
  Compare To Constant : simulink/Logic and Bit Operations/Compare To Constant  relop=>  const=pi  OutDataTypeStr=boolean
  Constant : Constant  Value=2*pi  OutDataTypeStr=single
  Multiply : Product
  Sign : Signum
  Subtract : Sum  Inputs=-+
  Switch : Switch  Criteria=u2 > Threshold
  psi_err_rad : Outport
  wires:
  Multiply/1 -> Switch/1
  Sign/1 -> Multiply/2
  Subtract/1 -> Multiply/1
  Constant/1 -> Subtract/1
  Switch/1 -> psi_err_rad/1
  Compare To Constant/1 -> Switch/2
  Abs/1 -> Compare To Constant/1, Subtract/2
  psi_err_in/1 -> Abs/1, Switch/3, Sign/1

== system FMS/FMS Commander/Commander/Arm/MC_Mode/Assist/Altitude/Heading Command/Controller/Move Control/DeadZone ==
  u : Inport
  Dead Zone : DeadZone  LowerValue=-th  UpperValue=th  SaturateOnIntegerOverflow=on
  Gain : Gain  Gain=1/(1-th)
  y : Outport
  wires:
  Gain/1 -> y/1
  Dead Zone/1 -> Gain/1
  u/1 -> Dead Zone/1

== system FMS/FMS Commander/Commander/Arm/MC_Mode/Assist/Altitude/Heading Command/Controller/Move Control/TD ==
  v : Inport
  Integrator : DiscreteIntegrator  SampleTime=-1  ICPrevOutput=DiscIntNeverNeededParam  ICPrevScaledInput=DiscIntNeverNeededParam
  Integrator1 : DiscreteIntegrator  SampleTime=-1  ICPrevOutput=DiscIntNeverNeededParam  ICPrevScaledInput=DiscIntNeverNeededParam
  Signal Copy : SignalConversion  OverrideOpt=off
  Subtract : Sum  Inputs=+-
  "fhan " : Subsystem  mask{r0=5*pi, h0=0.02}
      mask DialogControl ParameterGroupVar Prompt: fhan(v1,v2,r0,h0)
  v1 : Outport
  wires:
  "fhan "/1(fhan) -> Integrator/1
  Subtract/1 -> "fhan "/1(v1)
  Integrator/1 -> Integrator1/1, "fhan "/2(v2)  "v2"
  v/1 -> Subtract/2
  Integrator1/1 -> Subtract/1, Signal Copy/1
  Signal Copy/1 -> v1/1

== system FMS/FMS Commander/Commander/Arm/MC_Mode/Assist/Position/Altitude Command/Controller/Hold Control/Bus_Selection ==
  FMS_In : Inport
  Bus Selector2 : BusSelector  OutputSignals=INS_Out.h_R
  Gain : Gain  Gain=-1
  z_R_m : Outport
  wires:
  Gain/1 -> z_R_m/1
  Bus Selector2/1 -> Gain/1  "<h_R>"
  FMS_In/1 -> Bus Selector2/1

== system FMS/FMS Commander/Commander/Arm/MC_Mode/Assist/Position/Altitude Command/Controller/Move Control/Assist Land Speed ==
  u : Inport
  Gain : Gain  Gain=0.5
  Land_Speed : Constant  Value=FMS_PARAM.LAND_SPEED  OutDataTypeStr=single
  Min : MinMax  Inputs=2
  y : Outport
  wires:
  u/1 -> Min/2
  Land_Speed/1 -> Min/1
  Min/1 -> Gain/1
  Gain/1 -> y/1

== system FMS/FMS Commander/Commander/Arm/MC_Mode/Assist/Position/Altitude Command/Controller/Move Control/DeadZone ==
  u : Inport
  Dead Zone : DeadZone  LowerValue=-th  UpperValue=th  SaturateOnIntegerOverflow=on
  Gain : Gain  Gain=1/(1-th)
  y : Outport
  wires:
  Gain/1 -> y/1
  Dead Zone/1 -> Gain/1
  u/1 -> Dead Zone/1

== system FMS/FMS Commander/Commander/Arm/MC_Mode/Assist/Position/Heading Command/Controller/Hold Control/Bus_Selection ==
  FMS_In : Inport
  Bus Selector2 : BusSelector  OutputSignals=INS_Out.psi
  psi_rad : Outport
  wires:
  Bus Selector2/1 -> psi_rad/1  "<psi>"
  FMS_In/1 -> Bus Selector2/1

== system FMS/FMS Commander/Commander/Arm/MC_Mode/Assist/Position/Heading Command/Controller/Hold Control/psi_err_saturation ==
  psi_err_in : Inport
  Abs : Abs
  Compare To Constant : simulink/Logic and Bit Operations/Compare To Constant  relop=>  const=pi  OutDataTypeStr=boolean
  Constant : Constant  Value=2*pi  OutDataTypeStr=single
  Multiply : Product
  Sign : Signum
  Subtract : Sum  Inputs=-+
  Switch : Switch  Criteria=u2 > Threshold
  psi_err_rad : Outport
  wires:
  Multiply/1 -> Switch/1
  Sign/1 -> Multiply/2
  Subtract/1 -> Multiply/1
  Constant/1 -> Subtract/1
  Switch/1 -> psi_err_rad/1
  Compare To Constant/1 -> Switch/2
  Abs/1 -> Compare To Constant/1, Subtract/2
  psi_err_in/1 -> Abs/1, Switch/3, Sign/1

== system FMS/FMS Commander/Commander/Arm/MC_Mode/Assist/Position/Heading Command/Controller/Move Control/DeadZone ==
  u : Inport
  Dead Zone : DeadZone  LowerValue=-th  UpperValue=th  SaturateOnIntegerOverflow=on
  Gain : Gain  Gain=1/(1-th)
  y : Outport
  wires:
  Gain/1 -> y/1
  Dead Zone/1 -> Gain/1
  u/1 -> Dead Zone/1

== system FMS/FMS Commander/Commander/Arm/MC_Mode/Assist/Position/Heading Command/Controller/Move Control/TD ==
  v : Inport
  Integrator : DiscreteIntegrator  SampleTime=-1  ICPrevOutput=DiscIntNeverNeededParam  ICPrevScaledInput=DiscIntNeverNeededParam
  Integrator1 : DiscreteIntegrator  SampleTime=-1  ICPrevOutput=DiscIntNeverNeededParam  ICPrevScaledInput=DiscIntNeverNeededParam
  Signal Copy : SignalConversion  OverrideOpt=off
  Subtract : Sum  Inputs=+-
  "fhan " : Subsystem  mask{r0=5*pi, h0=0.02}
      mask DialogControl ParameterGroupVar Prompt: fhan(v1,v2,r0,h0)
  v1 : Outport
  wires:
  "fhan "/1(fhan) -> Integrator/1
  Subtract/1 -> "fhan "/1(v1)
  Integrator/1 -> Integrator1/1, "fhan "/2(v2)  "v2"
  v/1 -> Subtract/2
  Integrator1/1 -> Subtract/1, Signal Copy/1
  Signal Copy/1 -> v1/1

== system FMS/FMS Commander/Commander/Arm/MC_Mode/Assist/Position/Position Command/Controller/Hold Control/Bus_Selection ==
  FMS_In : Inport
  Bus Selector2 : BusSelector  OutputSignals=INS_Out.x_R,INS_Out.y_R
  Mux : Mux  Inputs=2
  xy_R_O_m : Outport
  wires:
  Bus Selector2/2 -> Mux/2  "<y_R>"
  Mux/1 -> xy_R_O_m/1
  Bus Selector2/1 -> Mux/1  "<x_R>"
  FMS_In/1 -> Bus Selector2/1

== system FMS/FMS Commander/Commander/Arm/MC_Mode/Assist/Position/Position Command/Controller/Move Control/DeadZone ==
  u : Inport
  Dead Zone : DeadZone  LowerValue=-th  UpperValue=th  SaturateOnIntegerOverflow=on
  Gain : Gain  Gain=1/(1-th)
  y : Outport
  wires:
  Gain/1 -> y/1
  Dead Zone/1 -> Gain/1
  u/1 -> Dead Zone/1

== system FMS/FMS Commander/Commander/Arm/MC_Mode/Assist/Position/Position Command/Controller/Move Control/DeadZone1 ==
  u : Inport
  Dead Zone : DeadZone  LowerValue=-th  UpperValue=th  SaturateOnIntegerOverflow=on
  Gain : Gain  Gain=1/(1-th)
  y : Outport
  wires:
  u/1 -> Dead Zone/1
  Dead Zone/1 -> Gain/1
  Gain/1 -> y/1

== system FMS/FMS Commander/Commander/Arm/MC_Mode/Assist/Position/Position Command/Controller/Move Control/TD ==
  v : Inport
  Integrator : DiscreteIntegrator  SampleTime=-1  ICPrevOutput=DiscIntNeverNeededParam  ICPrevScaledInput=DiscIntNeverNeededParam
  Integrator1 : DiscreteIntegrator  SampleTime=-1  ICPrevOutput=DiscIntNeverNeededParam  ICPrevScaledInput=DiscIntNeverNeededParam
  Signal Copy : SignalConversion  OverrideOpt=off
  Subtract : Sum  Inputs=+-
  "fhan " : Subsystem  mask{r0=4*9.806, h0=0.1}
      mask DialogControl ParameterGroupVar Prompt: fhan(v1,v2,r0,h0)
  v1 : Outport
  wires:
  "fhan "/1(fhan) -> Integrator/1
  Subtract/1 -> "fhan "/1(v1)
  Integrator/1 -> Integrator1/1, "fhan "/2(v2)  "v2"
  v/1 -> Subtract/2
  Integrator1/1 -> Subtract/1, Signal Copy/1
  Signal Copy/1 -> v1/1

== system FMS/FMS Commander/Commander/Arm/MC_Mode/Assist/Stabilize/Heading Command/Controller/Hold Control/Bus_Selection ==
  FMS_In : Inport
  Bus Selector2 : BusSelector  OutputSignals=INS_Out.psi
  psi_rad : Outport
  wires:
  Bus Selector2/1 -> psi_rad/1  "<psi>"
  FMS_In/1 -> Bus Selector2/1

== system FMS/FMS Commander/Commander/Arm/MC_Mode/Assist/Stabilize/Heading Command/Controller/Hold Control/psi_err_saturation ==
  psi_err_in : Inport
  Abs : Abs
  Compare To Constant : simulink/Logic and Bit Operations/Compare To Constant  relop=>  const=pi  OutDataTypeStr=boolean
  Constant : Constant  Value=2*pi  OutDataTypeStr=single
  Multiply : Product
  Sign : Signum
  Subtract : Sum  Inputs=-+
  Switch : Switch  Criteria=u2 > Threshold
  psi_err_rad : Outport
  wires:
  Multiply/1 -> Switch/1
  Sign/1 -> Multiply/2
  Subtract/1 -> Multiply/1
  Constant/1 -> Subtract/1
  Switch/1 -> psi_err_rad/1
  Compare To Constant/1 -> Switch/2
  Abs/1 -> Compare To Constant/1, Subtract/2
  psi_err_in/1 -> Abs/1, Switch/3, Sign/1

== system FMS/FMS Commander/Commander/Arm/MC_Mode/Assist/Stabilize/Heading Command/Controller/Move Control/DeadZone ==
  u : Inport
  Dead Zone : DeadZone  LowerValue=-th  UpperValue=th  SaturateOnIntegerOverflow=on
  Gain : Gain  Gain=1/(1-th)
  y : Outport
  wires:
  Gain/1 -> y/1
  Dead Zone/1 -> Gain/1
  u/1 -> Dead Zone/1

== system FMS/FMS Commander/Commander/Arm/MC_Mode/Assist/Stabilize/Heading Command/Controller/Move Control/TD ==
  v : Inport
  Integrator : DiscreteIntegrator  SampleTime=-1  ICPrevOutput=DiscIntNeverNeededParam  ICPrevScaledInput=DiscIntNeverNeededParam
  Integrator1 : DiscreteIntegrator  SampleTime=-1  ICPrevOutput=DiscIntNeverNeededParam  ICPrevScaledInput=DiscIntNeverNeededParam
  Signal Copy : SignalConversion  OverrideOpt=off
  Subtract : Sum  Inputs=+-
  "fhan " : Subsystem  mask{r0=5*pi, h0=0.02}
      mask DialogControl ParameterGroupVar Prompt: fhan(v1,v2,r0,h0)
  v1 : Outport
  wires:
  "fhan "/1(fhan) -> Integrator/1
  Subtract/1 -> "fhan "/1(v1)
  Integrator/1 -> Integrator1/1, "fhan "/2(v2)  "v2"
  v/1 -> Subtract/2
  Integrator1/1 -> Subtract/1, Signal Copy/1
  Signal Copy/1 -> v1/1

== system FMS/FMS Commander/Commander/Arm/MC_Mode/Auto/Mission/Mission_SubSystem/Heading Commander/Heading Control/Heading Control ==
  FMS_In : Inport
  psi_cmd_rad : Inport  Port=2
  Bus_Selection : Subsystem
  Gain2 : Gain  Gain=FMS_PARAM.YAW_P  OutDataTypeStr=single
  Saturation : Saturate  UpperLimit=FMS_PARAM.YAW_RATE_LIM  LowerLimit=-FMS_PARAM.YAW_RATE_LIM
  Sum : Sum  Inputs=-+|
  psi_saturation : Subsystem
  psi_rate_cmd_radPs : Outport
  wires:
  Saturation/1 -> psi_rate_cmd_radPs/1
  FMS_In/1 -> Bus_Selection/1(FMS_In)
  Sum/1 -> psi_saturation/1(psi_in)  "psi_error_rad"
  psi_saturation/1(psi_rad) -> Gain2/1
  Bus_Selection/1(psi_rad) -> Sum/1  "psi_est_rad"
  Gain2/1 -> Saturation/1
  psi_cmd_rad/1 -> Sum/2

== system FMS/FMS Commander/Commander/Arm/MC_Mode/Auto/Mission/Mission_SubSystem/Heading Commander/Heading Control/TD ==
  v : Inport
  v0 : Inport  Port=2
  Integrator : DiscreteIntegrator  SampleTime=-1  LimitOutput=on  UpperSaturationLimit=FMS_PARAM.YAW_RATE_LIM  LowerSaturationLimit=-FMS_PARAM.YAW_RATE_LIM  ICPrevOutput=DiscIntNeverNeededParam  ICPrevScaledInput=DiscIntNeverNeededParam
  Integrator1 : DiscreteIntegrator  InitialConditionSource=external  SampleTime=-1  ICPrevOutput=DiscIntNeverNeededParam  ICPrevScaledInput=DiscIntNeverNeededParam
  Subtract : Sum  Inputs=+-
  "fhan " : Subsystem  mask{r0=pi/4, h0=pi/4}
      mask DialogControl ParameterGroupVar Prompt: fhan(v1,v2,r0,h0)
  v1 : Outport
  wires:
  Integrator1/1 -> v1/1, Subtract/1
  v/1 -> Subtract/2
  Integrator/1 -> "fhan "/2(v2), Integrator1/1  "v2"
  Subtract/1 -> "fhan "/1(v1)
  "fhan "/1(fhan) -> Integrator/1
  v0/1 -> Integrator1/2

== system FMS/FMS Commander/Commander/Arm/MC_Mode/Auto/Mission/Mission_SubSystem/Heading Commander/Heading Control/psi_saturation ==
  psi_in : Inport
  Abs : Abs
  Add : Sum  Inputs=-+
  Compare To Constant : simulink/Logic and Bit Operations/Compare To Constant  relop=>  const=pi  OutDataTypeStr=boolean
  Constant : Constant  Value=2*pi  OutDataTypeStr=single
  Constant1 : Constant  Value=2*pi  OutDataTypeStr=single
  Multiply : Product
  Rem : Math  Operator=rem  SaturateOnIntegerOverflow=on
  Sign : Signum
  Switch : Switch  Criteria=u2 > Threshold
  psi_rad : Outport
  wires:
  Constant1/1 -> Rem/2
  psi_in/1 -> Rem/1
  Switch/1 -> psi_rad/1
  Sign/1 -> Multiply/2
  Constant/1 -> Multiply/1
  Multiply/1 -> Add/1
  Add/1 -> Switch/1
  Compare To Constant/1 -> Switch/2
  Abs/1 -> Compare To Constant/1
  Rem/1 -> Abs/1, Switch/3, Add/2, Sign/1

== system FMS/FMS Commander/Commander/Arm/MC_Mode/Auto/Mission/Mission_SubSystem/Heading Commander/Heading Control/psi_saturation1 ==
  psi_in : Inport
  Abs : Abs
  Add : Sum  Inputs=-+
  Compare To Constant : simulink/Logic and Bit Operations/Compare To Constant  relop=>  const=pi  OutDataTypeStr=boolean
  Constant : Constant  Value=2*pi  OutDataTypeStr=single
  Constant1 : Constant  Value=2*pi  OutDataTypeStr=single
  Multiply : Product
  Rem : Math  Operator=rem  SaturateOnIntegerOverflow=on
  Sign : Signum
  Switch : Switch  Criteria=u2 > Threshold
  psi_rad : Outport
  wires:
  Rem/1 -> Sign/1, Add/2, Switch/3, Abs/1
  Abs/1 -> Compare To Constant/1
  Compare To Constant/1 -> Switch/2
  Add/1 -> Switch/1
  Multiply/1 -> Add/1
  Constant/1 -> Multiply/1
  Sign/1 -> Multiply/2
  Switch/1 -> psi_rad/1
  psi_in/1 -> Rem/1
  Constant1/1 -> Rem/2

== system FMS/FMS Commander/Commander/Arm/MC_Mode/Auto/Mission/Mission_SubSystem/Velocity Commander/Altitude Control/Target Height ==
  FMS_In : Inport
  Add : Sum
  Bus Selector : BusSelector  OutputSignals=Cmd_In.sp_waypoint,Cmd_In.cur_waypoint
  Bus Selector1 : BusSelector  OutputSignals=INS_Out.x_R,INS_Out.y_R
  Bus Selector2 : BusSelector  OutputSignals=Cmd_In.cur_waypoint,Cmd_In.sp_waypoint
  Divide : Product  Inputs=*/
  Multiply : Product
  Mux : Mux  Inputs=2
  Saturation : Saturate  UpperLimit=1  LowerLimit=0
  Selector : Selector  InputPortWidth=3  IndexOptions=Index vector (dialog)  Indices=3  OutputSizes=1
  Selector1 : Selector  InputPortWidth=3  IndexOptions=Index vector (dialog)  Indices=3  OutputSizes=1
  Selector2 : Selector  InputPortWidth=3  IndexOptions=Index vector (dialog)  Indices=[1 2]  OutputSizes=1
  Selector3 : Selector  InputPortWidth=3  IndexOptions=Index vector (dialog)  Indices=[1 2]  OutputSizes=1
  Subtract : Sum  Inputs=+-
  Sum : Sum  Inputs=|+-
  Sum1 : Sum  Inputs=-+|
  Vector Modulus : FMT_Model_Lib/Math/Vector Modulus
      settings: SourceProductName=FMT Toolbox
  Vector Modulus1 : FMT_Model_Lib/Math/Vector Modulus
      settings: SourceProductName=FMT Toolbox
  h_R_sp : Outport
  wires:
  Multiply/1 -> Add/2
  Bus Selector1/1 -> Mux/1  "<x_R>"
  Bus Selector/1 -> Selector1/1  "<sp_waypoint>"
  Vector Modulus1/1 -> Divide/2
  Sum1/1 -> Vector Modulus1/1
  Sum/1 -> Vector Modulus/1
  Selector2/1 -> Sum1/1, Sum/2
  FMS_In/1 -> Bus Selector2/1, Bus Selector1/1, Bus Selector/1
  Bus Selector2/2 -> Selector3/1  "<sp_waypoint>"
  Vector Modulus/1 -> Divide/1
  Bus Selector1/2 -> Mux/2  "<y_R>"
  Bus Selector2/1 -> Selector2/1  "<cur_waypoint>"
  Selector1/1 -> Subtract/1
  Mux/1 -> Sum/1
  Subtract/1 -> Multiply/1
  Divide/1 -> Saturation/1
  Selector3/1 -> Sum1/2
  Bus Selector/2 -> Selector/1  "<cur_waypoint>"
  Selector/1 -> Add/1, Subtract/2
  Saturation/1 -> Multiply/2
  Add/1 -> h_R_sp/1

== system FMS/FMS Commander/Commander/Arm/MC_Mode/Auto/Mission/Mission_SubSystem/Velocity Commander/Hold Position/Altitude Hold ==
  FMS_In : Inport
  Controller : Subsystem
  Detect Movement : Subsystem
  w_cmd_mPs : Outport
  wires:
  Controller/1(w_cmd_mPs) -> w_cmd_mPs/1
  Detect Movement/1(motion_state) -> Controller/1(motion_state)
  FMS_In/1 -> Controller/2(FMS_In), Detect Movement/1(FMS_In)

== system FMS/FMS Commander/Commander/Arm/MC_Mode/Auto/Mission/Mission_SubSystem/Velocity Commander/Hold Position/Position Hold ==
  FMS_In : Inport
  Controller : Subsystem
  Demux : Demux  Outputs=2
  Detect Movement : Subsystem
  u_cmd_mPs : Outport
  v_cmd_mPs : Outport  Port=2
  wires:
  FMS_In/1 -> Controller/2(FMS_In), Detect Movement/1(FMS_In)
  Demux/2 -> v_cmd_mPs/1
  Demux/1 -> u_cmd_mPs/1
  Controller/1(uv_cmd_mPs) -> Demux/1
  Detect Movement/1(motion_state) -> Controller/1(motion_state)

== system FMS/FMS Commander/Commander/Arm/MC_Mode/Auto/Mission/Mission_SubSystem/Velocity Commander/Lateral Acceleration/Included Angle ==
  vec1 : Inport
  vec2 : Inport  Port=2
  2D Cross Product : FMT_Model_Lib/Math/2D Cross Product
      settings: SourceProductName=FMT Toolbox
  Acos : Trigonometry  Operator=acos
  Constant4 : Constant  OutDataTypeStr=single
  Demux : Demux  Outputs=2
  Demux1 : Demux  Outputs=2
  Dot Product : DotProduct  InputSameDT=on  OutDataTypeStr=Inherit: Inherit via internal rule
  Multiply : Product
  Mux : Mux  Inputs=2
  Mux1 : Mux  Inputs=2
  Sign1 : Signum
  Switch2 : Switch  Criteria=u2 ~= 0
  Vector Normalize : FMT_Model_Lib/Math/Vector Normalize
      settings: SourceProductName=FMT Toolbox
  Vector Normalize1 : FMT_Model_Lib/Math/Vector Normalize
      settings: SourceProductName=FMT Toolbox
  angle_rad : Outport
  wires:
  Switch2/1 -> Multiply/2
  Acos/1 -> Multiply/1
  Mux/1 -> Vector Normalize1/1
  vec2/1 -> Demux/1
  Constant4/1 -> Switch2/3
  Demux/1 -> Mux/2
  vec1/1 -> Demux1/1
  Multiply/1 -> angle_rad/1
  2D Cross Product/1 -> Sign1/1
  Vector Normalize/1 -> 2D Cross Product/2, Dot Product/1
  Demux/2 -> Mux/1
  Vector Normalize1/1 -> 2D Cross Product/1, Dot Product/2
  Sign1/1 -> Switch2/2, Switch2/1
  Demux1/2 -> Mux1/1
  Mux1/1 -> Vector Normalize/1
  Demux1/1 -> Mux1/2
  Dot Product/1 -> Acos/1

== system FMS/FMS Commander/Commander/Arm/MC_Mode/Auto/Mission/Mission_SubSystem/Velocity Commander/Lateral Acceleration To Speed/Ground Speed ==
  Vg : Inport
  p3p2 : Inport  Port=2
  Constant : Constant  Value=0  OutDataTypeStr=single
  Multiply2 : Product
  Mux : Mux  Inputs=2
  Vector Normalize2 : FMT_Model_Lib/Math/Vector Normalize
      settings: SourceProductName=FMT Toolbox
  Vg_O_cmd : Outport
  wires:
  Vg/1 -> Multiply2/2
  Constant/1 -> Mux/2
  Mux/1 -> Vector Normalize2/1
  p3p2/1 -> Mux/1
  Vector Normalize2/1 -> Multiply2/1
  Multiply2/1 -> Vg_O_cmd/1

== system FMS/FMS Commander/Commander/Arm/MC_Mode/Auto/Mission/Mission_SubSystem/Velocity Commander/Lateral Acceleration To Speed/Included Angle ==
  vec1 : Inport
  vec2 : Inport  Port=2
  Acos : Trigonometry  Operator=acos
  Constant4 : Constant  OutDataTypeStr=single
  Cross Product : FMT_Model_Lib/Math/2D Cross Product
      settings: SourceProductName=FMT Toolbox
  Demux : Demux  Outputs=2
  Demux1 : Demux  Outputs=2
  Dot Product : DotProduct  InputSameDT=on  OutDataTypeStr=Inherit: Inherit via internal rule
  Multiply : Product
  Mux : Mux  Inputs=2
  Mux1 : Mux  Inputs=2
  Sign1 : Signum
  Switch2 : Switch  Criteria=u2 ~= 0
  Vector Normalize : FMT_Model_Lib/Math/Vector Normalize
      settings: SourceProductName=FMT Toolbox
  Vector Normalize1 : FMT_Model_Lib/Math/Vector Normalize
      settings: SourceProductName=FMT Toolbox
  angle_rad : Outport
  wires:
  Switch2/1 -> Multiply/2
  Acos/1 -> Multiply/1
  Mux/1 -> Vector Normalize1/1
  vec2/1 -> Demux/1
  Constant4/1 -> Switch2/3
  Demux/1 -> Mux/2
  vec1/1 -> Demux1/1
  Multiply/1 -> angle_rad/1
  Cross Product/1 -> Sign1/1
  Vector Normalize/1 -> Cross Product/2, Dot Product/1
  Demux/2 -> Mux/1
  Vector Normalize1/1 -> Cross Product/1, Dot Product/2
  Sign1/1 -> Switch2/2, Switch2/1
  Demux1/2 -> Mux1/1
  Mux1/1 -> Vector Normalize/1
  Demux1/1 -> Mux1/2
  Dot Product/1 -> Acos/1

== system FMS/FMS Commander/Commander/Arm/MC_Mode/Auto/Mission/Mission_SubSystem/Velocity Commander/Lateral Acceleration To Speed/Rotation Matrix ==
  l1_omega : Inport
  psi : Inport  Port=2
  reset : Inport  Port=3  PortDimensions=1
  Add : Sum  Inputs=-+
  Discrete-Time Integrator : DiscreteIntegrator  ExternalReset=level  SampleTime=-1  StateName=l1_heading  ICPrevOutput=DiscIntNeverNeededParam  ICPrevScaledInput=DiscIntNeverNeededParam
  Psi To DCM : FMT_Model_Lib/Transformation/Psi To DCM
      settings: SourceProductName=FMT Toolbox
  M_CO : Outport
  wires:
  Add/1 -> Psi To DCM/1
  l1_omega/1 -> Discrete-Time Integrator/1  "l1_omega"
  psi/1 -> Add/2
  Discrete-Time Integrator/1 -> Add/1  "l1_psi"
  Psi To DCM/1 -> M_CO/1
  reset/1 -> Discrete-Time Integrator/2
